simulink model "frt_dqpll"  (R2026b)
settings: Solver=ode23tb  StopTime=param.sim.simlength  FixedStep=param.glb_time.tc  MaxStep=param.glb_time.tc
values from neighbouring files (symbols this model uses):
  param = struct()    [init_model.m]    (also in plotting_results_plls.m = evalin('base', 'param'))
undefined symbols (not defined in the file or in its folder): magnitude
libraries: fl_lib x45, nesl_utility x28, afe_uvw_ctrl x4, discrete_time_low_pass_filter x4, threephase_inductor_lib x1, three_phase_voltage_with_frt_emulator_mfcn x1, three_phase_pwm_modulator x1
(part 2 of 4)

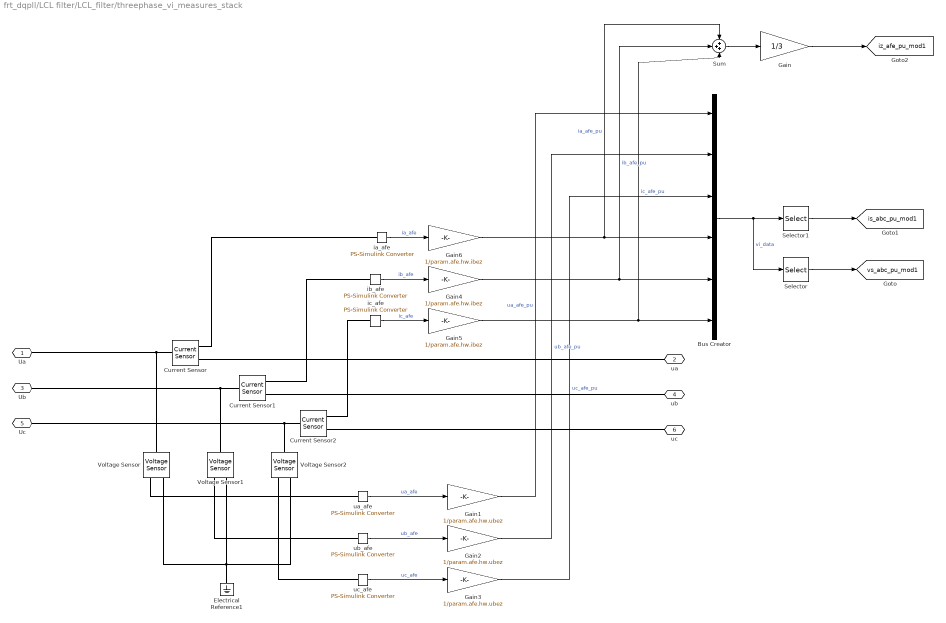
== system frt_dqpll/LCL filter/LCL_filter/threephase_vi_measures_stack ==
  Bus Creator : BusCreator  Inputs=6
  Current Sensor : fl_lib/Electrical/Electrical Sensors/Current Sensor
  Current Sensor1 : fl_lib/Electrical/Electrical Sensors/Current Sensor
  Current Sensor2 : fl_lib/Electrical/Electrical Sensors/Current Sensor
  Electrical Reference1 : fl_lib/Electrical/Electrical Elements/Electrical Reference
  Gain : Gain  Gain=1/3
  Gain1 : Gain  Gain=1/param.afe.hw.ubez
  Gain2 : Gain  Gain=1/param.afe.hw.ubez
  Gain3 : Gain  Gain=1/param.afe.hw.ubez
  Gain4 : Gain  Gain=1/param.afe.hw.ibez
  Gain5 : Gain  Gain=1/param.afe.hw.ibez
  Gain6 : Gain  Gain=1/param.afe.hw.ibez
  Selector : Selector  InputPortWidth=6  IndexOptions=Index vector (dialog)  Indices=[1 2 3]  OutputSizes=1  RuntimeRangeChecks=off
  Selector1 : Selector  InputPortWidth=6  IndexOptions=Index vector (dialog)  Indices=[4 5 6]  OutputSizes=1  RuntimeRangeChecks=off
  Sum : Sum  Inputs=+++
  Voltage Sensor : fl_lib/Electrical/Electrical Sensors/Voltage Sensor
  Voltage Sensor1 : fl_lib/Electrical/Electrical Sensors/Voltage Sensor
  Voltage Sensor2 : fl_lib/Electrical/Electrical Sensors/Voltage Sensor
  ia_afe : nesl_utility/PS-Simulink Converter  PhysicalDomain=network_engine_domain  SubClassName=ps_output  LeftPortType=input  RightPortType=output  PseudoPeriodic=off  Frequencies=[]  VectorFormat=1-D array  Unit=A  AffineConversion=off
  ib_afe : nesl_utility/PS-Simulink Converter  PhysicalDomain=network_engine_domain  SubClassName=ps_output  LeftPortType=input  RightPortType=output  PseudoPeriodic=off  Frequencies=[]  VectorFormat=1-D array  Unit=A  AffineConversion=off
  ic_afe : nesl_utility/PS-Simulink Converter  PhysicalDomain=network_engine_domain  SubClassName=ps_output  LeftPortType=input  RightPortType=output  PseudoPeriodic=off  Frequencies=[]  VectorFormat=1-D array  Unit=A  AffineConversion=off
  ua_afe : nesl_utility/PS-Simulink Converter  PhysicalDomain=network_engine_domain  SubClassName=ps_output  LeftPortType=input  RightPortType=output  PseudoPeriodic=off  Frequencies=[]  VectorFormat=1-D array  Unit=V  AffineConversion=off
  ub_afe : nesl_utility/PS-Simulink Converter  PhysicalDomain=network_engine_domain  SubClassName=ps_output  LeftPortType=input  RightPortType=output  PseudoPeriodic=off  Frequencies=[]  VectorFormat=1-D array  Unit=V  AffineConversion=off
  uc_afe : nesl_utility/PS-Simulink Converter  PhysicalDomain=network_engine_domain  SubClassName=ps_output  LeftPortType=input  RightPortType=output  PseudoPeriodic=off  Frequencies=[]  VectorFormat=1-D array  Unit=V  AffineConversion=off
  Ua : PMIOPort  Side=Left
  ua : PMIOPort  Port=2  Side=Right
  Ub : PMIOPort  Port=3  Side=Left
  ub : PMIOPort  Port=4  Side=Right
  Uc : PMIOPort  Port=5  Side=Left
  uc : PMIOPort  Port=6  Side=Right
  tag scope: is_abc_pu_mod1=global, iz_afe_pu_mod1=global, vs_abc_pu_mod1=global
  wires:
  Bus Creator/1 -> Selector/1, Selector1/1  "vi_data"
  Selector/1 -> [vs_abc_pu_mod1]
  ib_afe/1 -> Gain4/1  "ib_afe"
  ia_afe/1 -> Gain6/1  "ia_afe"
  ic_afe/1 -> Gain5/1  "ic_afe"
  ua_afe/1 -> Gain1/1  "ua_afe"
  ub_afe/1 -> Gain2/1  "ub_afe"
  uc_afe/1 -> Gain3/1  "uc_afe"
  Selector1/1 -> [is_abc_pu_mod1]
  Sum/1 -> Gain/1
  Gain/1 -> [iz_afe_pu_mod1]
  Gain1/1 -> Bus Creator/1  "ua_afe_pu"
  Gain2/1 -> Bus Creator/2  "ub_afe_pu"
  Gain3/1 -> Bus Creator/3  "uc_afe_pu"
  Gain6/1 -> Sum/1, Bus Creator/4  "ia_afe_pu"
  Gain4/1 -> Sum/2, Bus Creator/5  "ib_afe_pu"
  Gain5/1 -> Bus Creator/6, Sum/3  "ic_afe_pu"
  connections:
  Current Sensor1/LConn1 -- Ub/RConn1 -- Voltage Sensor1/LConn1
  Electrical Reference1/LConn1 -- Voltage Sensor/RConn2 -- Voltage Sensor2/RConn2 -- Voltage Sensor1/RConn2
  Voltage Sensor/RConn1 -- ua_afe/LConn1
  Current Sensor/RConn2 -- ua/RConn1
  Voltage Sensor1/RConn1 -- ub_afe/LConn1
  Voltage Sensor2/LConn1 -- Uc/RConn1 -- Current Sensor2/LConn1
  Current Sensor/LConn1 -- Ua/RConn1 -- Voltage Sensor/LConn1
  Current Sensor1/RConn2 -- ub/RConn1
  Voltage Sensor2/RConn1 -- uc_afe/LConn1
  ib_afe/LConn1 -- Current Sensor1/RConn1
  ia_afe/LConn1 -- Current Sensor/RConn1
  ic_afe/LConn1 -- Current Sensor2/RConn1
  Current Sensor2/RConn2 -- uc/RConn1

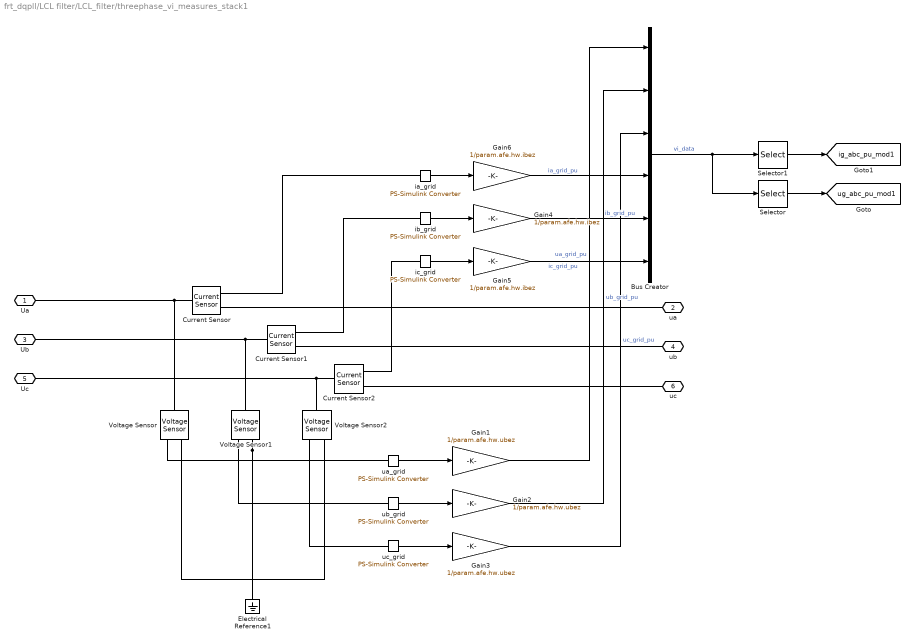
== system frt_dqpll/LCL filter/LCL_filter/threephase_vi_measures_stack1 ==
  Bus Creator : BusCreator  Inputs=6
  Current Sensor : fl_lib/Electrical/Electrical Sensors/Current Sensor
  Current Sensor1 : fl_lib/Electrical/Electrical Sensors/Current Sensor
  Current Sensor2 : fl_lib/Electrical/Electrical Sensors/Current Sensor
  Electrical Reference1 : fl_lib/Electrical/Electrical Elements/Electrical Reference
  Gain1 : Gain  Gain=1/param.afe.hw.ubez
  Gain2 : Gain  Gain=1/param.afe.hw.ubez
  Gain3 : Gain  Gain=1/param.afe.hw.ubez
  Gain4 : Gain  Gain=1/param.afe.hw.ibez
  Gain5 : Gain  Gain=1/param.afe.hw.ibez
  Gain6 : Gain  Gain=1/param.afe.hw.ibez
  Selector : Selector  InputPortWidth=6  IndexOptions=Index vector (dialog)  Indices=[1 2 3]  OutputSizes=1  RuntimeRangeChecks=off
  Selector1 : Selector  InputPortWidth=6  IndexOptions=Index vector (dialog)  Indices=[4 5 6]  OutputSizes=1  RuntimeRangeChecks=off
  Voltage Sensor : fl_lib/Electrical/Electrical Sensors/Voltage Sensor
  Voltage Sensor1 : fl_lib/Electrical/Electrical Sensors/Voltage Sensor
  Voltage Sensor2 : fl_lib/Electrical/Electrical Sensors/Voltage Sensor
  ia_grid : nesl_utility/PS-Simulink Converter  PhysicalDomain=network_engine_domain  SubClassName=ps_output  LeftPortType=input  RightPortType=output  PseudoPeriodic=off  Frequencies=[]  VectorFormat=1-D array  Unit=A  AffineConversion=off
  ib_grid : nesl_utility/PS-Simulink Converter  PhysicalDomain=network_engine_domain  SubClassName=ps_output  LeftPortType=input  RightPortType=output  PseudoPeriodic=off  Frequencies=[]  VectorFormat=1-D array  Unit=A  AffineConversion=off
  ic_grid : nesl_utility/PS-Simulink Converter  PhysicalDomain=network_engine_domain  SubClassName=ps_output  LeftPortType=input  RightPortType=output  PseudoPeriodic=off  Frequencies=[]  VectorFormat=1-D array  Unit=A  AffineConversion=off
  ua_grid : nesl_utility/PS-Simulink Converter  PhysicalDomain=network_engine_domain  SubClassName=ps_output  LeftPortType=input  RightPortType=output  PseudoPeriodic=off  Frequencies=[]  VectorFormat=1-D array  Unit=V  AffineConversion=off
  ub_grid : nesl_utility/PS-Simulink Converter  PhysicalDomain=network_engine_domain  SubClassName=ps_output  LeftPortType=input  RightPortType=output  PseudoPeriodic=off  Frequencies=[]  VectorFormat=1-D array  Unit=V  AffineConversion=off
  uc_grid : nesl_utility/PS-Simulink Converter  PhysicalDomain=network_engine_domain  SubClassName=ps_output  LeftPortType=input  RightPortType=output  PseudoPeriodic=off  Frequencies=[]  VectorFormat=1-D array  Unit=V  AffineConversion=off
  Ua : PMIOPort  Side=Left
  ua : PMIOPort  Port=2  Side=Right
  Ub : PMIOPort  Port=3  Side=Left
  ub : PMIOPort  Port=4  Side=Right
  Uc : PMIOPort  Port=5  Side=Left
  uc : PMIOPort  Port=6  Side=Right
  tag scope: ig_abc_pu_mod1=global, ug_abc_pu_mod1=global
  wires:
  Selector1/1 -> [ig_abc_pu_mod1]
  uc_grid/1 -> Gain3/1
  ub_grid/1 -> Gain2/1
  ua_grid/1 -> Gain1/1
  ic_grid/1 -> Gain5/1
  ia_grid/1 -> Gain6/1
  ib_grid/1 -> Gain4/1
  Selector/1 -> [ug_abc_pu_mod1]
  Bus Creator/1 -> Selector1/1, Selector/1  "vi_data"
  Gain1/1 -> Bus Creator/1  "ua_grid_pu"
  Gain2/1 -> Bus Creator/2  "ub_grid_pu"
  Gain3/1 -> Bus Creator/3  "uc_grid_pu"
  Gain6/1 -> Bus Creator/4  "ia_grid_pu"
  Gain4/1 -> Bus Creator/5  "ib_grid_pu"
  Gain5/1 -> Bus Creator/6  "ic_grid_pu"
  connections:
  Current Sensor2/RConn2 -- uc/RConn1
  ic_grid/LConn1 -- Current Sensor2/RConn1
  ia_grid/LConn1 -- Current Sensor/RConn1
  ib_grid/LConn1 -- Current Sensor1/RConn1
  Voltage Sensor2/RConn1 -- uc_grid/LConn1
  Current Sensor1/RConn2 -- ub/RConn1
  Voltage Sensor/LConn1 -- Current Sensor/LConn1 -- Ua/RConn1
  Current Sensor2/LConn1 -- Voltage Sensor2/LConn1 -- Uc/RConn1
  Voltage Sensor1/RConn1 -- ub_grid/LConn1
  Current Sensor/RConn2 -- ua/RConn1
  Voltage Sensor/RConn1 -- ua_grid/LConn1
  Voltage Sensor1/RConn2 -- Voltage Sensor2/RConn2 -- Voltage Sensor/RConn2 -- Electrical Reference1/LConn1
  Voltage Sensor1/LConn1 -- Current Sensor1/LConn1 -- Ub/RConn1

== system frt_dqpll/grid/grid_emulator/3ph_Dyg_ssc ==
  Electrical Reference1 : fl_lib/Electrical/Electrical Elements/Electrical Reference
  PS Terminator : fl_lib/Physical Signals/Sinks/PS Terminator
  PS Terminator1 : fl_lib/Physical Signals/Sinks/PS Terminator
  PS Terminator2 : fl_lib/Physical Signals/Sinks/PS Terminator
  configurable_trafo : SimscapeComponentBlock  Description=Configurable transformer: one or two three-phase primaries (star or delta), secondary three-phase (star or delta, any clock number) or single-phase (turns distribution ws) on a three-limb core. Component configurable_transformer.configurable_transformer (pwr-control/library, foundation/electrical_machines/+configurable_transformer).  SourceFile=configurable_transformer.configurable_transformer  ComponentPath=configurable_transformer.configurable_transformer  ComponentVariants="[\"configurable_transformer.configurable_transformer\"]"  ComponentVariantNames="[\"configurable_transformer\"]"  ClassName=configurable_transformer  SchemaVersion=1  primaries=configurable_transformer.n_primaries.one  conn1=configurable_transformer.connection.delta  conn2=configurable_transformer.connection.star  clock2=0  secondary=configurable_transformer.secondary_winding.star  clock3=param.grid.emu.trafo.pu.clock3  ws=[1, -1, 0]  Sr=param.grid.emu.trafo.pwr_nom A*V  V1=param.grid.emu.trafo.u1_nom V  V2=400 V  V3=param.grid.emu.trafo.u2_nom V  fr=param.grid.emu.trafo.f_nom Hz  r1=param.grid.emu.trafo.pu.r1  l1=param.grid.emu.trafo.pu.l1  r2=0.005  l2=0.030  r3=param.grid.emu.trafo.pu.r3  l3=param.grid.emu.trafo.pu.l3  lm=param.grid.emu.trafo.pu.lm  lm0=param.grid.emu.trafo.pu.lm0  rfe=param.grid.emu.trafo.pu.rfe  i1a_specify=off  i1a_priority=None  i1a=0 A  i1a_nominal_specify=off  i1a_nominal_value=1  i1a_nominal_unit=A  i1b_specify=off  i1b_priority=None  i1b=0 A  i1b_nominal_specify=off  i1b_nominal_value=1  i1b_nominal_unit=A  i1c_specify=off  i1c_priority=None  i1c=0 A  i1c_nominal_specify=off  i1c_nominal_value=1  i1c_nominal_unit=A  i2a_specify=off  i2a_priority=None  i2a=0 A  i2a_nominal_specify=off  i2a_nominal_value=1  i2a_nominal_unit=A  i2b_specify=off  i2b_priority=None  i2b=0 A  i2b_nominal_specify=off  i2b_nominal_value=1  i2b_nominal_unit=A  i2c_specify=off  i2c_priority=None  i2c=0 A  i2c_nominal_specify=off  i2c_nominal_value=1  i2c_nominal_unit=A  i3a_specify=off  i3a_priority=None  i3a=0 A  i3a_nominal_specify=off  i3a_nominal_value=1  i3a_nominal_unit=A  i3b_specify=off  i3b_priority=None  i3b=0 A  i3b_nominal_specify=off  i3b_nominal_value=1  i3b_nominal_unit=A  i3c_specify=off  i3c_priority=None  i3c=0 A  i3c_nominal_specify=off  i3c_nominal_value=1  i3c_nominal_unit=A  i3_specify=off  i3_priority=None  i3=0 A  i3_nominal_specify=off  i3_nominal_value=1  i3_nominal_unit=A
      settings: CopyFcn=simscape.sscblock.internal.componentBlockCallback(gcbh,'COPY')  PreCopyFcn=simscape.sscblock.internal.componentBlockCallback(gcbh,'PRECOPY')  PreDeleteFcn=simscape.sscblock.internal.componentBlockCallback(gcbh,'PREDELETE')
      mask Type: Configurable Transformer
  ua : PMIOPort  Side=Right
  ub : PMIOPort  Port=2  Side=Right
  uc : PMIOPort  Port=3  Side=Right
  Ua : PMIOPort  Port=4  Side=Left
  Ub : PMIOPort  Port=5  Side=Left
  Uc : PMIOPort  Port=6  Side=Left
  connections:
  Uc/RConn1 -- configurable_trafo/LConn3
  configurable_trafo/LConn2 -- Ub/RConn1
  configurable_trafo/RConn1 -- ua/RConn1
  configurable_trafo/LConn1 -- Ua/RConn1
  ub/RConn1 -- configurable_trafo/RConn2
  configurable_trafo/RConn3 -- uc/RConn1
  Electrical Reference1/LConn1 -- configurable_trafo/RConn4
  PS Terminator/LConn1 -- configurable_trafo/RConn5
  PS Terminator1/LConn1 -- configurable_trafo/RConn6
  configurable_trafo/RConn7 -- PS Terminator2/LConn1

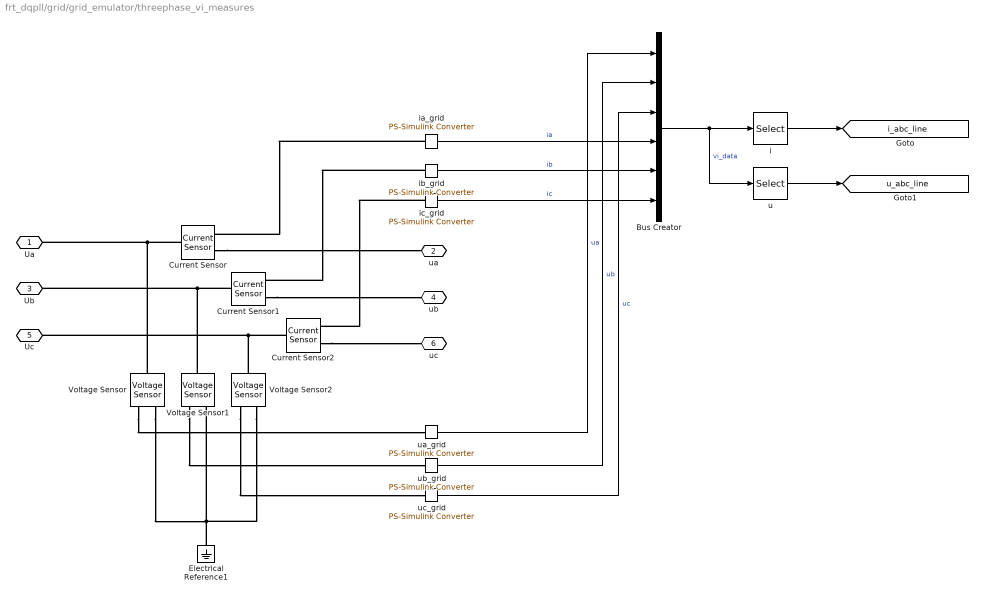
== system frt_dqpll/grid/grid_emulator/threephase_vi_measures ==
  Bus Creator : BusCreator  Inputs=6
  Current Sensor : fl_lib/Electrical/Electrical Sensors/Current Sensor
  Current Sensor1 : fl_lib/Electrical/Electrical Sensors/Current Sensor
  Current Sensor2 : fl_lib/Electrical/Electrical Sensors/Current Sensor
  Electrical Reference1 : fl_lib/Electrical/Electrical Elements/Electrical Reference
  Voltage Sensor : fl_lib/Electrical/Electrical Sensors/Voltage Sensor
  Voltage Sensor1 : fl_lib/Electrical/Electrical Sensors/Voltage Sensor
  Voltage Sensor2 : fl_lib/Electrical/Electrical Sensors/Voltage Sensor
  i : Selector  InputPortWidth=6  IndexOptions=Index vector (dialog)  Indices=[4 5 6]  OutputSizes=1  RuntimeRangeChecks=off
  ia_grid : nesl_utility/PS-Simulink Converter  PhysicalDomain=network_engine_domain  SubClassName=ps_output  LeftPortType=input  RightPortType=output  PseudoPeriodic=off  Frequencies=[]  VectorFormat=1-D array  Unit=A  AffineConversion=off
  ib_grid : nesl_utility/PS-Simulink Converter  PhysicalDomain=network_engine_domain  SubClassName=ps_output  LeftPortType=input  RightPortType=output  PseudoPeriodic=off  Frequencies=[]  VectorFormat=1-D array  Unit=A  AffineConversion=off
  ic_grid : nesl_utility/PS-Simulink Converter  PhysicalDomain=network_engine_domain  SubClassName=ps_output  LeftPortType=input  RightPortType=output  PseudoPeriodic=off  Frequencies=[]  VectorFormat=1-D array  Unit=A  AffineConversion=off
  u : Selector  InputPortWidth=6  IndexOptions=Index vector (dialog)  Indices=[1 2 3]  OutputSizes=1  RuntimeRangeChecks=off
  ua_grid : nesl_utility/PS-Simulink Converter  PhysicalDomain=network_engine_domain  SubClassName=ps_output  LeftPortType=input  RightPortType=output  PseudoPeriodic=off  Frequencies=[]  VectorFormat=1-D array  Unit=V  AffineConversion=off
  ub_grid : nesl_utility/PS-Simulink Converter  PhysicalDomain=network_engine_domain  SubClassName=ps_output  LeftPortType=input  RightPortType=output  PseudoPeriodic=off  Frequencies=[]  VectorFormat=1-D array  Unit=V  AffineConversion=off
  uc_grid : nesl_utility/PS-Simulink Converter  PhysicalDomain=network_engine_domain  SubClassName=ps_output  LeftPortType=input  RightPortType=output  PseudoPeriodic=off  Frequencies=[]  VectorFormat=1-D array  Unit=V  AffineConversion=off
  Ua : PMIOPort  Side=Left
  ua : PMIOPort  Port=2  Side=Right
  Ub : PMIOPort  Port=3  Side=Left
  ub : PMIOPort  Port=4  Side=Right
  Uc : PMIOPort  Port=5  Side=Left
  uc : PMIOPort  Port=6  Side=Right
  tag scope: i_abc_line=global, u_abc_line=global
  wires:
  Bus Creator/1 -> i/1, u/1  "vi_data"
  ib_grid/1 -> Bus Creator/5  "ib"
  ia_grid/1 -> Bus Creator/4  "ia"
  ic_grid/1 -> Bus Creator/6  "ic"
  ua_grid/1 -> Bus Creator/1  "ua"
  ub_grid/1 -> Bus Creator/2  "ub"
  uc_grid/1 -> Bus Creator/3  "uc"
  i/1 -> [i_abc_line]
  u/1 -> [u_abc_line]
  connections:
  Current Sensor1/LConn1 -- Ub/RConn1 -- Voltage Sensor1/LConn1
  Electrical Reference1/LConn1 -- Voltage Sensor/RConn2 -- Voltage Sensor2/RConn2 -- Voltage Sensor1/RConn2
  Voltage Sensor/RConn1 -- ua_grid/LConn1
  Current Sensor/RConn2 -- ua/RConn1
  Voltage Sensor1/RConn1 -- ub_grid/LConn1
  Voltage Sensor2/LConn1 -- Current Sensor2/LConn1 -- Uc/RConn1
  Current Sensor/LConn1 -- Ua/RConn1 -- Voltage Sensor/LConn1
  Current Sensor1/RConn2 -- ub/RConn1
  Voltage Sensor2/RConn1 -- uc_grid/LConn1
  ib_grid/LConn1 -- Current Sensor1/RConn1
  ia_grid/LConn1 -- Current Sensor/RConn1
  ic_grid/LConn1 -- Current Sensor2/RConn1
  Current Sensor2/RConn2 -- uc/RConn1

== system frt_dqpll/AFE_control1/afe_control/FRT-VDE4110/positive_reactive_current_reference ==
  Step : Step  Time=param.afe.ref.time_i_react_pos_ref_1  InitialValue=param.afe.ref.i_react_pos_ref_1  FinalValue=param.afe.ref.i_react_pos_ref_2
  Step1 : Step  Time=param.afe.ref.time_i_react_pos_ref_2  FinalValue=param.afe.ref.i_react_pos_ref_3-param.afe.ref.i_react_pos_ref_2
  Sum7 : Sum  Inputs=|++
  i_react_pos_ref : Outport
  wires:
  Sum7/1 -> i_react_pos_ref/1
  Step1/1 -> Sum7/2
  Step/1 -> Sum7/1

== system frt_dqpll/AFE_control1/afe_control/grid_voltage_phase_lock_loops/DDSRF-PLL ==
  ug_abc_pu : Inport
  pll_stageA : Subsystem
  pll_stageB : Subsystem
  gamma_grid_ddsrf_pll : Outport
  omega_grid_ddsrf_pll : Outport  Port=2
  wires:
  pll_stageB/1(phase_grid_ddsrf_pll) -> pll_stageA/1(gamma_grid), gamma_grid_ddsrf_pll/1
  pll_stageA/2(u_grid_pos_eta) -> pll_stageB/2(u_grid_pos_eta)  "u_grid_pos_eta"
  pll_stageA/1(u_grid_pos_xi) -> pll_stageB/1(u_grid_pos_xi)  "u_grid_pos_xi"
  pll_stageB/2(omega_grid_ddsrf_pll) -> omega_grid_ddsrf_pll/1
  ug_abc_pu/1 -> pll_stageA/2(ug_abc_pu)

== system frt_dqpll/AFE_control1/afe_control/grid_voltage_phase_lock_loops/FHT-PLL ==
  ug_abc_pu : Inport
  pll_stageA : Subsystem
  pll_stageB : Subsystem
  gamma_grid_fht_pll : Outport
  omega_grid_fht_pll : Outport  Port=2
  wires:
  ug_abc_pu/1 -> pll_stageA/2(ug_abc_pu)
  pll_stageB/2(omega_grid_ddsrf_pll) -> omega_grid_fht_pll/1
  pll_stageA/1(u_grid_xi) -> pll_stageB/1(u_grid_pos_xi)  "u_grid_pos_xi"
  pll_stageA/2(u_grid_eta) -> pll_stageB/2(u_grid_pos_eta)  "u_grid_pos_eta"
  pll_stageB/1(gamma_grid_ddsrf_pll) -> gamma_grid_fht_pll/1, pll_stageA/1(gamma_grid)

== system frt_dqpll/AFE_control1/afe_control/grid_voltage_phase_lock_loops/dq_pll ==
  ug_abc_pu : Inport
  pll_stageA : Subsystem
  pll_stageB : Subsystem
  phase_grid_dqpll : Outport
  omega_grid_pu_dqpll : Outport  Port=2
  wires:
  pll_stageA/2(u_grid_pos_eta) -> pll_stageB/2(u_grid_pos_eta)  "u_grid_pos_eta"
  pll_stageB/1(phase_grid_pll) -> phase_grid_dqpll/1, pll_stageA/1(phase_grid)
  pll_stageA/1(u_grid_pos_xi) -> pll_stageB/1(u_grid_pos_xi)  "u_grid_pos_xi"
  pll_stageB/2(omega_grid_pu_pll) -> omega_grid_pu_dqpll/1
  ug_abc_pu/1 -> pll_stageA/2(ug_abc)

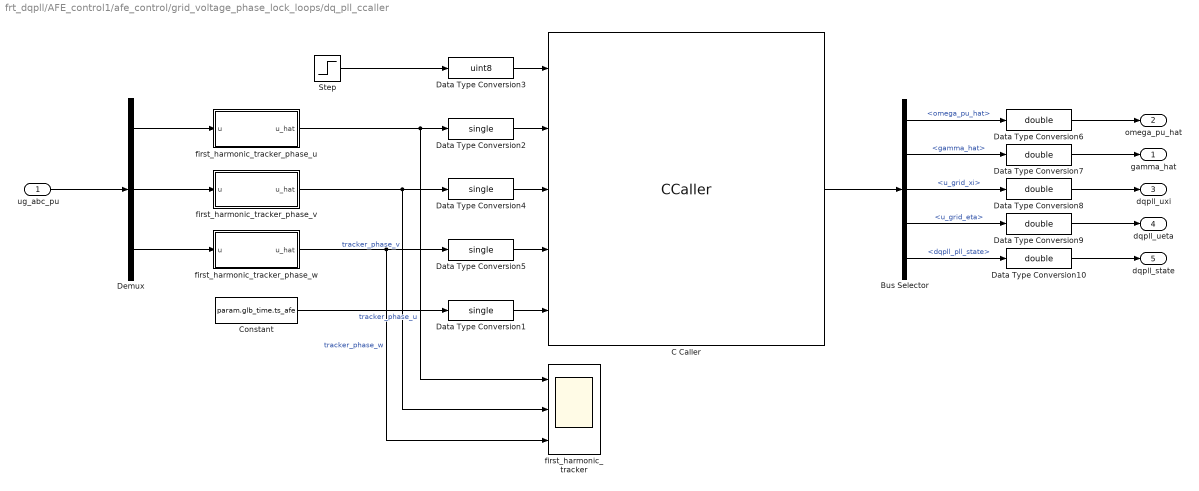
== system frt_dqpll/AFE_control1/afe_control/grid_voltage_phase_lock_loops/dq_pll_ccaller ==
  ug_abc_pu : Inport
  Bus Selector : BusSelector  OutputSignals=omega_pu_hat,gamma_hat,u_grid_xi,u_grid_eta,dqpll_pll_state
  C Caller : CCaller  FunctionName=dqpll_grid_process_simulink  PortSpecificationStruct="%)30     .    N H   8    (     @         %    \"     8    !     0         %  0 \"0    $    _    07)G3F%M90  4&]R=$YA;64 4V-O<&4     26YD97@     5'EP90      4VEZ90      27-';&]B86P   X    P    !@    @    $          4    (     0    ,    !         !   P!O=70 #@   #     &    \"     0         !0    @    !     P    $         $  # &]U=  .    .     8    (    !          %    \"     $    &     0         0   ...(+3319 chars)"
  Constant : Constant  Value=param.glb_time.ts_afe
  Data Type Conversion{1..2,4..5} (4 alike) : DataTypeConversion  OutDataTypeStr=single  SaturateOnIntegerOverflow=off  RndMeth=Floor
  Data Type Conversion{6..10} (5 alike) : DataTypeConversion  OutDataTypeStr=double  SaturateOnIntegerOverflow=off  RndMeth=Floor
  Data Type Conversion3 : DataTypeConversion  OutDataTypeStr=uint8  SaturateOnIntegerOverflow=off  RndMeth=Floor
  Demux : Demux  Outputs=3
  Step : Step  Time=0.01  InitialValue=1  FinalValue=0
  first_harmonic_tracker : Scope  NumInputPorts=3
      settings: ActiveDisplayYMinimum=-1.7184470891952515  ActiveDisplayYMaximum=1.8384636640548706
  first_harmonic_tracker_phase_u : Subsystem
  first_harmonic_tracker_phase_v : Subsystem
  first_harmonic_tracker_phase_w : Subsystem
  gamma_hat : Outport  VectorParamsAs1DForOutWhenUnconnected=off
  omega_pu_hat : Outport  Port=2  VectorParamsAs1DForOutWhenUnconnected=off
  dqpll_uxi : Outport  Port=3  VectorParamsAs1DForOutWhenUnconnected=off
  dqpll_ueta : Outport  Port=4  VectorParamsAs1DForOutWhenUnconnected=off
  dqpll_state : Outport  Port=5  VectorParamsAs1DForOutWhenUnconnected=off
  wires:
  Step/1 -> Data Type Conversion3/1
  Constant/1 -> Data Type Conversion1/1
  Data Type Conversion3/1 -> C Caller/1
  Data Type Conversion2/1 -> C Caller/2
  Data Type Conversion4/1 -> C Caller/3
  Data Type Conversion5/1 -> C Caller/4
  Data Type Conversion1/1 -> C Caller/5
  C Caller/1 -> Bus Selector/1
  Bus Selector/1 -> Data Type Conversion6/1  "<omega_pu_hat>"
  Bus Selector/2 -> Data Type Conversion7/1  "<gamma_hat>"
  Bus Selector/3 -> Data Type Conversion8/1  "<u_grid_xi>"
  Bus Selector/4 -> Data Type Conversion9/1  "<u_grid_eta>"
  Bus Selector/5 -> Data Type Conversion10/1  "<dqpll_pll_state>"
  Data Type Conversion7/1 -> gamma_hat/1
  Data Type Conversion10/1 -> dqpll_state/1
  Data Type Conversion8/1 -> dqpll_uxi/1
  Data Type Conversion9/1 -> dqpll_ueta/1
  ug_abc_pu/1 -> Demux/1
  Demux/1 -> first_harmonic_tracker_phase_u/1(u)
  Demux/2 -> first_harmonic_tracker_phase_v/1(u)
  Demux/3 -> first_harmonic_tracker_phase_w/1(u)
  Data Type Conversion6/1 -> omega_pu_hat/1
  first_harmonic_tracker_phase_u/1(u_hat) -> first_harmonic_tracker/1, Data Type Conversion2/1  "tracker_phase_u"
  first_harmonic_tracker_phase_v/1(u_hat) -> first_harmonic_tracker/2, Data Type Conversion4/1  "tracker_phase_v"
  first_harmonic_tracker_phase_w/1(u_hat) -> first_harmonic_tracker/3, Data Type Conversion5/1  "tracker_phase_w"

== system frt_dqpll/AFE_control1/afe_control/ig afe quantizzation and one step delay/ig afe quantizzation and one step delay ==
  ig_u_pu : Inport
  ig_v_pu : Inport  Port=2
  ig_w_pu : Inport  Port=3
  Gain4 : Gain  Gain=-1
  Gain5 : Gain  Gain=-1
  Gain6 : Gain  Gain=-1
  Quantizer1 : Quantizer  QuantizationInterval=param.meas.adc_quantization
  Quantizer2 : Quantizer  QuantizationInterval=param.meas.adc_quantization
  Quantizer4 : Quantizer  QuantizationInterval=param.meas.adc_quantization
  Unit Delay : UnitDelay  SampleTime=-1
  Unit Delay1 : UnitDelay  SampleTime=-1
  Unit Delay2 : UnitDelay  SampleTime=-1
  Zero-Order Hold : ZeroOrderHold  SampleTime=-1
  Zero-Order Hold1 : ZeroOrderHold  SampleTime=-1
  Zero-Order Hold2 : ZeroOrderHold  SampleTime=-1
  igd_u_pu : Outport
  igd_v_pu : Outport  Port=2
  igd_w_pu : Outport  Port=3
  wires:
  Quantizer1/1 -> Unit Delay1/1
  Quantizer4/1 -> Unit Delay/1
  Quantizer2/1 -> Unit Delay2/1
  ig_u_pu/1 -> Zero-Order Hold/1
  ig_v_pu/1 -> Zero-Order Hold1/1
  ig_w_pu/1 -> Zero-Order Hold2/1
  Unit Delay/1 -> Gain4/1
  Unit Delay1/1 -> Gain5/1
  Unit Delay2/1 -> Gain6/1
  Gain4/1 -> igd_u_pu/1
  Gain5/1 -> igd_v_pu/1
  Gain6/1 -> igd_w_pu/1
  Zero-Order Hold/1 -> Quantizer4/1
  Zero-Order Hold1/1 -> Quantizer1/1
  Zero-Order Hold2/1 -> Quantizer2/1

== system frt_dqpll/AFE_control1/afe_control/is afe quantizzation and one step delay/is afe quantizzation and one step delay ==
  is_u_pu : Inport
  is_v_pu : Inport  Port=2
  is_w_pu : Inport  Port=3
  Quantizer : Quantizer  QuantizationInterval=param.meas.adc_quantization
  Quantizer1 : Quantizer  QuantizationInterval=param.meas.adc_quantization
  Quantizer2 : Quantizer  QuantizationInterval=param.meas.adc_quantization
  Unit Delay : UnitDelay  SampleTime=-1
  Unit Delay1 : UnitDelay  SampleTime=-1
  Unit Delay2 : UnitDelay  SampleTime=-1
  Zero-Order Hold : ZeroOrderHold  SampleTime=-1
  Zero-Order Hold1 : ZeroOrderHold  SampleTime=-1
  Zero-Order Hold2 : ZeroOrderHold  SampleTime=-1
  isd_u_pu : Outport
  isd_v_pu : Outport  Port=2
  isd_w_pu : Outport  Port=3
  wires:
  Unit Delay/1 -> isd_u_pu/1
  Unit Delay1/1 -> isd_v_pu/1
  Unit Delay2/1 -> isd_w_pu/1
  Quantizer/1 -> Unit Delay/1
  Quantizer1/1 -> Unit Delay1/1
  Quantizer2/1 -> Unit Delay2/1
  is_u_pu/1 -> Zero-Order Hold/1
  is_v_pu/1 -> Zero-Order Hold1/1
  is_w_pu/1 -> Zero-Order Hold2/1
  Zero-Order Hold/1 -> Quantizer/1
  Zero-Order Hold1/1 -> Quantizer1/1
  Zero-Order Hold2/1 -> Quantizer2/1

== system frt_dqpll/AFE_control1/afe_control/ug afe quantizzation and one step delay/ug afe quantizzation and one step delay ==
  ug_u_pu : Inport
  ug_v_pu : Inport  Port=2
  ug_w_pu : Inport  Port=3
  Quantizer1 : Quantizer  QuantizationInterval=param.meas.adc_quantization
  Quantizer2 : Quantizer  QuantizationInterval=param.meas.adc_quantization
  Quantizer4 : Quantizer  QuantizationInterval=param.meas.adc_quantization
  Unit Delay : UnitDelay  SampleTime=-1
  Unit Delay1 : UnitDelay  SampleTime=-1
  Unit Delay2 : UnitDelay  SampleTime=-1
  Zero-Order Hold : ZeroOrderHold  SampleTime=-1
  Zero-Order Hold1 : ZeroOrderHold  SampleTime=-1
  Zero-Order Hold2 : ZeroOrderHold  SampleTime=-1
  ugd_u_pu : Outport
  ugd_v_pu : Outport  Port=2
  ugd_w_pu : Outport  Port=3
  wires:
  Unit Delay/1 -> ugd_u_pu/1
  Unit Delay1/1 -> ugd_v_pu/1
  Unit Delay2/1 -> ugd_w_pu/1
  Quantizer4/1 -> Unit Delay/1
  Quantizer1/1 -> Unit Delay1/1
  Quantizer2/1 -> Unit Delay2/1
  ug_w_pu/1 -> Zero-Order Hold2/1
  ug_v_pu/1 -> Zero-Order Hold1/1
  ug_u_pu/1 -> Zero-Order Hold/1
  Zero-Order Hold/1 -> Quantizer4/1
  Zero-Order Hold1/1 -> Quantizer1/1
  Zero-Order Hold2/1 -> Quantizer2/1

== system frt_dqpll/AFE_control1/afe_control/grid_voltage_phase_lock_loops/DDSRF-PLL/pll_stageA ==
  gamma_grid : Inport
  ug_abc_pu : Inport  Port=2
  Demux : Demux  Outputs=3
  Math Function : Math  Operator=magnitude^2  SignedPower=on
  Math Function1 : Math  Operator=magnitude^2  SignedPower=on
  Reciprocal Sqrt : Sqrt  Operator=rSqrt
  Saturation : Saturate  UpperLimit=inf  LowerLimit=0.02
  Sum : Sum  Inputs=|++
  filter_and_transformation : Subsystem
  sequences : Subsystem
  u_grid_pos_xi : Outport  VectorParamsAs1DForOutWhenUnconnected=off
  u_grid_pos_eta : Outport  Port=2  VectorParamsAs1DForOutWhenUnconnected=off
  tag scope: Vgrid_unorm_ddsrf=scoped
  wires:
  Saturation/1 -> Reciprocal Sqrt/1
  Reciprocal Sqrt/1 -> [Vgrid_unorm_ddsrf]
  Sum/1 -> Saturation/1
  Math Function1/1 -> Sum/2
  Math Function/1 -> Sum/1
  filter_and_transformation/2(ug_beta) -> Math Function1/1, sequences/2(u_grid_beta)
  filter_and_transformation/1(ug_alpha) -> Math Function/1, sequences/1(u_grid_alpha)
  Demux/3 -> filter_and_transformation/3(ug_c)
  Demux/2 -> filter_and_transformation/2(ug_b)
  Demux/1 -> filter_and_transformation/1(ug_a)
  ug_abc_pu/1 -> Demux/1
  sequences/1(u_grid_pos_xi) -> u_grid_pos_xi/1
  sequences/2(u_grid_pos_eta) -> u_grid_pos_eta/1
  gamma_grid/1 -> sequences/3(phase_angle)

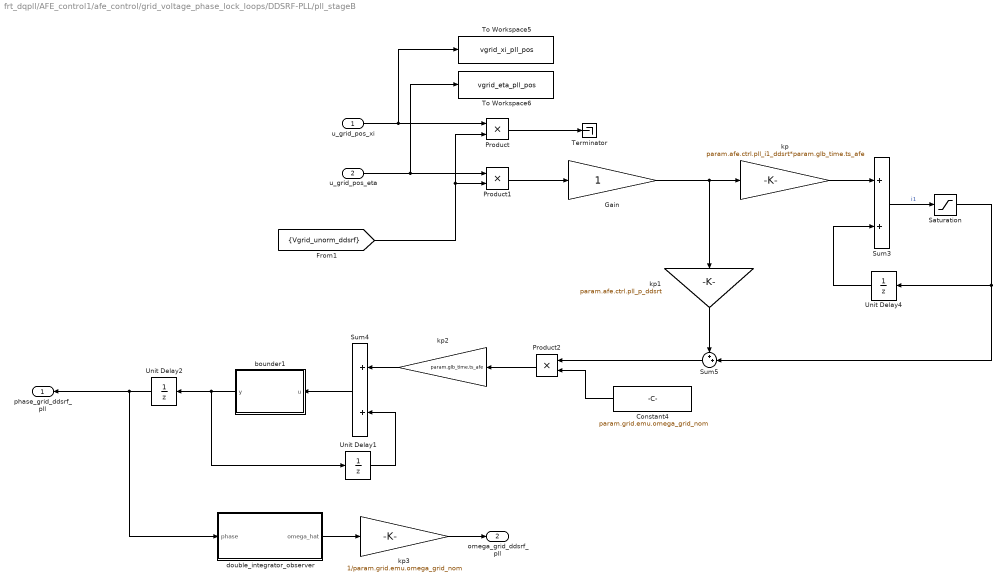
== system frt_dqpll/AFE_control1/afe_control/grid_voltage_phase_lock_loops/DDSRF-PLL/pll_stageB ==
  u_grid_pos_xi : Inport
  u_grid_pos_eta : Inport  Port=2
  Constant4 : Constant  Value=param.grid.emu.omega_grid_nom
  Gain : Gain
  Product : Product  RndMeth=Zero
  Product1 : Product  RndMeth=Zero
  Product2 : Product  RndMeth=Zero
  Saturation : Saturate  UpperLimit=1.5  LowerLimit=0.5
  Sum3 : Sum  SaturateOnIntegerOverflow=on
  Sum4 : Sum  SaturateOnIntegerOverflow=on
  Sum5 : Sum  Inputs=++|
  Terminator : Terminator
  To Workspace5 : ToWorkspace  VariableName=vgrid_xi_pll_pos  SampleTime=-1
      settings: MaxDataPoints=param.glb_time.Ns_afe
  To Workspace6 : ToWorkspace  VariableName=vgrid_eta_pll_pos  SampleTime=-1
      settings: MaxDataPoints=param.glb_time.Ns_afe
  Unit Delay1 : UnitDelay  SampleTime=-1
  Unit Delay2 : UnitDelay  SampleTime=-1
  Unit Delay4 : UnitDelay  SampleTime=-1
  bounder1 : MATLAB Function  TreatAsAtomicUnit=on
  double_integrator_observer : Subsystem
  kp : Gain  Gain=param.afe.ctrl.pll_i1_ddsrt*param.glb_time.ts_afe  SaturateOnIntegerOverflow=on  OutDataTypeStr=Inherit: Same as input  ParamDataTypeStr=Inherit: Same as input
  kp1 : Gain  Gain=param.afe.ctrl.pll_p_ddsrt  SaturateOnIntegerOverflow=on  OutDataTypeStr=Inherit: Same as input  ParamDataTypeStr=Inherit: Same as input
  kp2 : Gain  Gain=param.glb_time.ts_afe  SaturateOnIntegerOverflow=on  OutDataTypeStr=Inherit: Same as input  ParamDataTypeStr=Inherit: Same as input
  kp3 : Gain  Gain=1/param.grid.emu.omega_grid_nom  SaturateOnIntegerOverflow=on  OutDataTypeStr=Inherit: Same as input  ParamDataTypeStr=Inherit: Same as input
  phase_grid_ddsrf_pll : Outport  VectorParamsAs1DForOutWhenUnconnected=off
  omega_grid_ddsrf_pll : Outport  Port=2  VectorParamsAs1DForOutWhenUnconnected=off
  wires:
  Unit Delay2/1 -> double_integrator_observer/1(phase), phase_grid_ddsrf_pll/1
  kp1/1 -> Sum5/1
  Product2/1 -> kp2/1
  u_grid_pos_eta/1 -> Product1/1, To Workspace6/1
  u_grid_pos_xi/1 -> To Workspace5/1, Product/1
  bounder1/1(y) -> Unit Delay1/1, Unit Delay2/1
  Sum5/1 -> Product2/1
  kp/1 -> Sum3/1
  [Vgrid_unorm_ddsrf] -> Product1/2, Product/2
  Constant4/1 -> Product2/2
  kp2/1 -> Sum4/1
  Sum3/1 -> Saturation/1  "i1"
  Unit Delay1/1 -> Sum4/2
  Sum4/1 -> bounder1/1(u)
  Unit Delay4/1 -> Sum3/2
  double_integrator_observer/1(omega_hat) -> kp3/1
  Product/1 -> Terminator/1
  kp3/1 -> omega_grid_ddsrf_pll/1
  Product1/1 -> Gain/1
  Gain/1 -> kp1/1, kp/1
  Saturation/1 -> Unit Delay4/1, Sum5/2

== system frt_dqpll/AFE_control1/afe_control/grid_voltage_phase_lock_loops/FHT-PLL/pll_stageA ==
  gamma_grid : Inport
  ug_abc_pu : Inport  Port=2
  Demux : Demux  Outputs=3
  Math Function : Math  Operator=magnitude^2  SignedPower=on
  Math Function1 : Math  Operator=magnitude^2  SignedPower=on
  Reciprocal Sqrt : Sqrt  Operator=rSqrt
  Saturation : Saturate  UpperLimit=inf  LowerLimit=0.02
  Sum : Sum  Inputs=|++
  filter_and_transformation : Subsystem
  sequences : Subsystem
  u_grid_xi : Outport  VectorParamsAs1DForOutWhenUnconnected=off
  u_grid_eta : Outport  Port=2  VectorParamsAs1DForOutWhenUnconnected=off
  tag scope: Vgrid_unorm_fht=scoped
  wires:
  gamma_grid/1 -> sequences/3(phase_angle)
  sequences/2(u_grid_eta) -> u_grid_eta/1
  sequences/1(u_grid_xi) -> u_grid_xi/1
  ug_abc_pu/1 -> Demux/1
  Demux/1 -> filter_and_transformation/1(ug_a)
  Demux/2 -> filter_and_transformation/2(ug_b)
  Demux/3 -> filter_and_transformation/3(ug_c)
  filter_and_transformation/1(ug_alpha) -> Math Function/1, sequences/1(u_grid_alpha)
  filter_and_transformation/2(ug_beta) -> Math Function1/1, sequences/2(u_grid_beta)
  Math Function/1 -> Sum/1
  Math Function1/1 -> Sum/2
  Sum/1 -> Saturation/1
  Reciprocal Sqrt/1 -> [Vgrid_unorm_fht]
  Saturation/1 -> Reciprocal Sqrt/1

== system frt_dqpll/AFE_control1/afe_control/grid_voltage_phase_lock_loops/FHT-PLL/pll_stageB ==
  u_grid_pos_xi : Inport
  u_grid_pos_eta : Inport  Port=2
  Constant4 : Constant  Value=param.grid.emu.omega_grid_nom
  Gain : Gain  Gain=-1
  Product : Product  RndMeth=Zero
  Product1 : Product  RndMeth=Zero
  Product2 : Product  RndMeth=Zero
  Sum3 : Sum  SaturateOnIntegerOverflow=on
  Sum4 : Sum  SaturateOnIntegerOverflow=on
  Sum5 : Sum  Inputs=++|
  Terminator : Terminator
  Unit Delay1 : UnitDelay  SampleTime=-1
  Unit Delay2 : UnitDelay  SampleTime=-1
  Unit Delay4 : UnitDelay  SampleTime=-1
  bounder1 : MATLAB Function  TreatAsAtomicUnit=on
  double_integrator_observer : Subsystem
  kp : Gain  Gain=param.afe.ctrl.pll_i1_fht*param.glb_time.ts_afe  SaturateOnIntegerOverflow=on  OutDataTypeStr=Inherit: Same as input  ParamDataTypeStr=Inherit: Same as input
  kp1 : Gain  Gain=param.afe.ctrl.pll_p_fht  SaturateOnIntegerOverflow=on  OutDataTypeStr=Inherit: Same as input  ParamDataTypeStr=Inherit: Same as input
  kp2 : Gain  Gain=param.glb_time.ts_afe  SaturateOnIntegerOverflow=on  OutDataTypeStr=Inherit: Same as input  ParamDataTypeStr=Inherit: Same as input
  kp3 : Gain  Gain=1/param.grid.emu.omega_grid_nom  SaturateOnIntegerOverflow=on  OutDataTypeStr=Inherit: Same as input  ParamDataTypeStr=Inherit: Same as input
  gamma_grid_ddsrf_pll : Outport  VectorParamsAs1DForOutWhenUnconnected=off
  omega_grid_ddsrf_pll : Outport  Port=2  VectorParamsAs1DForOutWhenUnconnected=off
  wires:
  Gain/1 -> kp/1, kp1/1
  Product1/1 -> Gain/1
  kp3/1 -> omega_grid_ddsrf_pll/1
  Product/1 -> Terminator/1
  double_integrator_observer/1(omega_hat) -> kp3/1
  Unit Delay4/1 -> Sum3/2
  Sum4/1 -> bounder1/1(u)
  Unit Delay1/1 -> Sum4/2
  Sum3/1 -> Sum5/2, Unit Delay4/1  "i1"
  kp2/1 -> Sum4/1
  Constant4/1 -> Product2/2
  [Vgrid_unorm_fht] -> Product/2, Product1/2
  kp/1 -> Sum3/1
  Sum5/1 -> Product2/1
  bounder1/1(y) -> Unit Delay2/1, Unit Delay1/1
  u_grid_pos_xi/1 -> Product/1
  u_grid_pos_eta/1 -> Product1/1
  Product2/1 -> kp2/1
  kp1/1 -> Sum5/1
  Unit Delay2/1 -> double_integrator_observer/1(theta), gamma_grid_ddsrf_pll/1

== system frt_dqpll/AFE_control1/afe_control/grid_voltage_phase_lock_loops/dq_pll/pll_stageA ==
  phase_grid : Inport
  ug_abc : Inport  Port=2
  Demux : Demux  Outputs=3
  Math Function : Math  Operator=magnitude^2  SignedPower=on
  Math Function1 : Math  Operator=magnitude^2  SignedPower=on
  Reciprocal Sqrt : Sqrt  Operator=rSqrt
  Saturation : Saturate  UpperLimit=inf  LowerLimit=0.02
  Sum : Sum  Inputs=|++
  mormalization_and_transformation : Subsystem
  sequences : Subsystem
  u_grid_pos_xi : Outport  VectorParamsAs1DForOutWhenUnconnected=off
  u_grid_pos_eta : Outport  Port=2  VectorParamsAs1DForOutWhenUnconnected=off
  tag scope: Vgrid_unorm_dqpll=scoped
  wires:
  ug_abc/1 -> Demux/1
  Demux/1 -> mormalization_and_transformation/1(ug_a)
  Demux/2 -> mormalization_and_transformation/2(ug_b)
  Demux/3 -> mormalization_and_transformation/3(ug_c)
  phase_grid/1 -> sequences/3(gamma_grid)
  sequences/1(u_grid_pos_xi) -> u_grid_pos_xi/1
  sequences/2(u_grid_pos_eta) -> u_grid_pos_eta/1
  Math Function1/1 -> Sum/2
  mormalization_and_transformation/1(ug_alpha) -> Math Function/1, sequences/1(u_grid_alpha)
  mormalization_and_transformation/2(ug_beta) -> Math Function1/1, sequences/2(u_grid_beta)
  Reciprocal Sqrt/1 -> [Vgrid_unorm_dqpll]
  Sum/1 -> Saturation/1
  Math Function/1 -> Sum/1
  Saturation/1 -> Reciprocal Sqrt/1

== system frt_dqpll/AFE_control1/afe_control/grid_voltage_phase_lock_loops/dq_pll/pll_stageB ==
  u_grid_pos_xi : Inport
  u_grid_pos_eta : Inport  Port=2
  -2<x<2 : Saturate  UpperLimit=2  LowerLimit=-2
  Constant4 : Constant  Value=param.grid.emu.omega_grid_nom
  Gain : Gain  Gain=1/param.grid.emu.omega_grid_nom
  Product1 : Product  RndMeth=Zero
  Product2 : Product  RndMeth=Zero
  Sum3 : Sum  SaturateOnIntegerOverflow=on
  Sum4 : Sum  SaturateOnIntegerOverflow=on
  Sum5 : Sum  Inputs=++|
  Terminator : Terminator
  Unit Delay1 : UnitDelay  SampleTime=-1
  Unit Delay2 : UnitDelay  SampleTime=-1
  Unit Delay4 : UnitDelay  SampleTime=-1
  bounder1 : MATLAB Function  TreatAsAtomicUnit=on
  double_integrator_observer : Subsystem
  kp : Gain  Gain=param.afe.ctrl.pll_i1*param.glb_time.ts_afe  SaturateOnIntegerOverflow=on  OutDataTypeStr=Inherit: Same as input  ParamDataTypeStr=Inherit: Same as input
  kp2 : Gain  Gain=param.glb_time.ts_afe  SaturateOnIntegerOverflow=on  OutDataTypeStr=Inherit: Same as input  ParamDataTypeStr=Inherit: Same as input
  scheduled-p-gain : Subsystem
      settings: PortSchema="{\"entries\":[{\"content\":{\"sides\":[{\"content\":{},\"type\":\"ConnectorPlacement.EquallySpacedRectSide\",\"uuid\":\"88e64df2-a299-4c1b-9bac-7a615cd04a00\"},{\"content\":{\"side\":\"RIGHT\"},\"type\":\"ConnectorPlacement.EquallySpacedRectSide\",\"uuid\":\"ef1d7318-b0e2-4e96-bf99-c42bb4ec5202\"},{\"content\":{\"connectorIds\":[\"In1\"],\"side\":\"TOP\"},\"type\":\"ConnectorPlacement.EquallySpacedRectSide\",\"uuid\":\"96582c59-f6c8-40f1-b3cf-394cc239c4b2\"},{\"content\":{\"connectorIds\":[\"Out1\"],\"side\":\"BOTTOM\"},\"type\":\"ConnectorPlacement.EquallySpacedRectSide\",\"uuid\":\"9ac5cd0d-958f-4b67-b4ea-90856a0aa038\"}]},\"type\":\"ConnectorPlacement.EquallySpacedConnector\",\"uuid\":\"ca37db80-6b94-4315-bd9c-66307567cd1f\"}],\"packageUris\":[\"http://schema.mathworks.com/mf0/Connector/R2020b\"],\"version\":\"1.0\"}"
  phase_grid_pll : Outport  VectorParamsAs1DForOutWhenUnconnected=off
  omega_grid_pu_pll : Outport  Port=2  VectorParamsAs1DForOutWhenUnconnected=off
  wires:
  Unit Delay4/1 -> Sum3/2
  Sum3/1 -> -2<x<2/1
  Sum4/1 -> bounder1/1(u)
  Unit Delay1/1 -> Sum4/2
  -2<x<2/1 -> Sum5/2, Unit Delay4/1  "i1"
  kp2/1 -> Sum4/1
  Constant4/1 -> Product2/2
  [Vgrid_unorm_dqpll] -> Product1/2
  kp/1 -> Sum3/1
  Sum5/1 -> Product2/1
  bounder1/1(y) -> Unit Delay1/1, Unit Delay2/1
  u_grid_pos_eta/1 -> Product1/1
  Product2/1 -> kp2/1
  Product1/1 -> scheduled-p-gain/1(In1), kp/1
  scheduled-p-gain/1(Out2) -> Sum5/1
  Unit Delay2/1 -> double_integrator_observer/1(phase), phase_grid_pll/1
  double_integrator_observer/1(omega_hat) -> Gain/1
  Gain/1 -> omega_grid_pu_pll/1
  u_grid_pos_xi/1 -> Terminator/1

== system frt_dqpll/AFE_control1/afe_control/grid_voltage_phase_lock_loops/dq_pll_ccaller/first_harmonic_tracker_phase_u ==
  u : Inport
  Bus Selector : BusSelector  OutputSignals=output_pu_hat
  C Caller : CCaller  FunctionName=first_harmonic_tracker_process_simulink  PortSpecificationStruct="%)30     .    B \\   8    (     @         %    \"     D    !     0         %  0 \"0    $    _    07)G3F%M90  4&]R=$YA;64 4V-O<&4     26YD97@     5'EP90      4VEZ90      27-';&]B86P   X    P    !@    @    $          4    (     0    ,    !         !   P!O=70 #@   #     &    \"     0         !0    @    !     P    $         $  # &]U=  .    .     8    (    !          %    \"     $    &     0         0  ...(+4988 chars)"
  Constant : Constant  Value=param.glb_time.ts_afe
  Constant1 : Constant  Value=0
  Constant4 : Constant  Value=param.afe.ctrl.fht_grid.omega_fht
  Constant5 : Constant  Value=param.afe.ctrl.fht_grid.delta_fht
  Constant6 : Constant  Value=param.afe.ctrl.fht_grid.Ld_fht(1)
  Constant7 : Constant  Value=param.afe.ctrl.fht_grid.Ld_fht(2)
  Data Type Conversion{1..2,6..9} (6 alike) : DataTypeConversion  OutDataTypeStr=single  SaturateOnIntegerOverflow=off  RndMeth=Floor
  Data Type Conversion3 : DataTypeConversion  OutDataTypeStr=uint8  SaturateOnIntegerOverflow=off  RndMeth=Floor
  Data Type Conversion4 : DataTypeConversion  OutDataTypeStr=double  SaturateOnIntegerOverflow=off  RndMeth=Floor
  Data Type Conversion5 : DataTypeConversion  OutDataTypeStr=uint8  SaturateOnIntegerOverflow=off  RndMeth=Floor
  Step : Step  Time=0.0125  InitialValue=1  FinalValue=0
  u_hat : Outport
  wires:
  Data Type Conversion4/1 -> u_hat/1
  Data Type Conversion3/1 -> C Caller/1
  Data Type Conversion1/1 -> C Caller/3
  Data Type Conversion2/1 -> C Caller/2
  C Caller/1 -> Bus Selector/1
  Bus Selector/1 -> Data Type Conversion4/1  "<output_pu_hat>"
  Step/1 -> Data Type Conversion3/1
  u/1 -> Data Type Conversion2/1
  Constant/1 -> Data Type Conversion1/1
  Constant1/1 -> Data Type Conversion5/1
  Constant4/1 -> Data Type Conversion6/1
  Constant6/1 -> Data Type Conversion8/1
  Constant7/1 -> Data Type Conversion9/1
  Constant5/1 -> Data Type Conversion7/1
  Data Type Conversion5/1 -> C Caller/8
  Data Type Conversion6/1 -> C Caller/4
  Data Type Conversion7/1 -> C Caller/5
  Data Type Conversion8/1 -> C Caller/6
  Data Type Conversion9/1 -> C Caller/7
